simulink model "cars"  (Simulink 9.2)
settings: Solver=VariableStepAuto  StartTime=0  StopTime=100  FixedStep=0.1  MinStep=0.01  RelTol=1e-3  AbsTol=1e-5  EnableMultiTasking=on
settings Model: Creator=yoriyuki  LastModifiedBy=yoriyuki
settings SolverCC: AutoInsertRateTranBlk=on
settings DataIOCC: ExternalInput=[Throttle, Brake]  FinalStateName=SavePoint  InitialState=SavePoint  LimitDataPoints=off  SaveCompleteFinalSimState=on  SaveFormat=Dataset  SignalLoggingSaveFormat=Dataset  SaveOutput=off  SaveTime=off  StateSaveName=x  TimeSaveName=t  OutputSaveName=y
settings DebuggingCC: UnderspecifiedInitializationDetection=Simplified  MergeDetectMultiDrivingBlocksExec=error  FcnCallInpInsideContextMsg=error  AllowSymbolicDim=off  StateNameClashWarn=none
settings HardwareCC: ProdBitPerPointer=64  ProdBitPerSizeT=64  ProdBitPerPtrDiffT=64  ProdLargestAtomicFloat=Float  ProdIntDivRoundTo=Zero  ProdEndianess=LittleEndian  ProdWordSize=64  ProdHWDeviceType=Intel->x86-64 (Windows64)
settings ModelReferenceCC: PropagateSignalLabelsOutOfModel=on
settings GRTTargetCC: GeneratePreprocessorConditionals=Use local settings  CombineOutputUpdateFcns=on  GRTInterface=off
settings ConfigComp: CovShowResultsExplorer=off

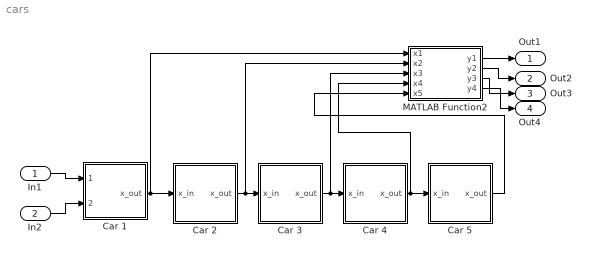
== system cars ==
  In1 : Inport
  In2 : Inport  Port=2
  Car 1 : Stateflow chart  TreatAsAtomicUnit=on
  Car 2 : Stateflow chart  TreatAsAtomicUnit=on
  Car 3 : Stateflow chart  TreatAsAtomicUnit=on
  Car 4 : Stateflow chart  TreatAsAtomicUnit=on
  Car 5 : Stateflow chart  TreatAsAtomicUnit=on
  MATLAB Function2 : MATLAB Function  TreatAsAtomicUnit=on
  Out1 : Outport
  Out2 : Outport  Port=2
  Out3 : Outport  Port=3
  Out4 : Outport  Port=4
  wires:
  Car 1/1(x_out) -> MATLAB Function2/1(x1), Car 2/1(x_in)
  Car 2/1(x_out) -> MATLAB Function2/2(x2), Car 3/1(x_in)
  Car 3/1(x_out) -> MATLAB Function2/3(x3), Car 4/1(x_in)
  Car 4/1(x_out) -> MATLAB Function2/4(x4), Car 5/1(x_in)
  Car 5/1(x_out) -> MATLAB Function2/5(x5)
  MATLAB Function2/1(y1) -> Out1/1
  MATLAB Function2/2(y2) -> Out2/1
  MATLAB Function2/3(y3) -> Out3/1
  MATLAB Function2/4(y4) -> Out4/1
  In1/1 -> Car 1/1(Throttle)
  In2/1 -> Car 1/2(Brake)

== stateflow chart Car 1 ==
  settings: updateMethod=CONTINUOUS
  state Run
    during:
    v_dot = -Throttle - Brake * v;
    x_dot = v;
    x_out = x;
  (default) -> Run
  data: Throttle input double; Brake input double; x local double =0; x_out output double; v local double =0
  data x settings: updateMethod=SF_CONTINUOUS_TIME_DATA
  data v settings: updateMethod=SF_CONTINUOUS_TIME_DATA

== stateflow chart Car 3 ==
  settings: updateMethod=CONTINUOUS
  state Chasing
    during:
    v_dot = 1;
    x_dot = -v;
    x_out = x;
  state Keeping
    during:
    x_dot = v;
    x_out = x;
  state Braking
    during:
    v_dot = -v;
    x_dot = -v;
    x_out = x;
  (default) -> Keeping
  Chasing -> Keeping : [x - x_in <= 10]
      | % [transition condition]{action}
  Keeping -> Chasing [order 1] : [x - x_in >=15]
  Braking -> Chasing : [x - x_in >= 20]
  Keeping -> Braking [order 2] : [x - x_in <=5]
  data: x_out output double; x local double =20; v local double =0; x_in input double
  data x settings: updateMethod=SF_CONTINUOUS_TIME_DATA
  data v settings: updateMethod=SF_CONTINUOUS_TIME_DATA
  data x_in settings: updateMethod=SF_CONTINUOUS_TIME_DATA

== stateflow chart Car 2 ==
  settings: updateMethod=CONTINUOUS
  state Chasing
    during:
    v_dot = 1;
    x_dot = -v;
    x_out = x;
  state Keeping
    during:
    x_dot = v;
    x_out = x;
  state Braking
    during:
    v_dot = -v;
    x_dot = -v;
    x_out = x;
  (default) -> Keeping
  Chasing -> Keeping : [x - x_in <= 10]
      | % [transition condition]{action}
  Keeping -> Chasing [order 1] : [x - x_in >=15]
  Braking -> Chasing : [x - x_in >= 20]
  Keeping -> Braking [order 2] : [x - x_in <=5]
  data: x_out output double; x local double =10; v local double =0; x_in input double
  data x settings: updateMethod=SF_CONTINUOUS_TIME_DATA
  data v settings: updateMethod=SF_CONTINUOUS_TIME_DATA
  data x_in settings: updateMethod=SF_CONTINUOUS_TIME_DATA

== stateflow chart Car 4 ==
  settings: updateMethod=CONTINUOUS
  state Chasing
    during:
    v_dot = 1;
    x_dot = -v;
    x_out = x;
  state Keeping
    during:
    x_dot = v;
    x_out = x;
  state Braking
    during:
    v_dot = -v;
    x_dot = -v;
    x_out = x;
  (default) -> Keeping
  Chasing -> Keeping : [x - x_in <= 10]
      | % [transition condition]{action}
  Keeping -> Chasing [order 1] : [x - x_in >=15]
  Braking -> Chasing : [x - x_in >= 20]
  Keeping -> Braking [order 2] : [x - x_in <=5]
  data: x_out output double; x local double =30; v local double =0; x_in input double
  data x settings: updateMethod=SF_CONTINUOUS_TIME_DATA
  data v settings: updateMethod=SF_CONTINUOUS_TIME_DATA
  data x_in settings: updateMethod=SF_CONTINUOUS_TIME_DATA

== stateflow chart Car 5 ==
  settings: updateMethod=CONTINUOUS
  state Keeping
    during:
    x_dot = v;
    x_out = x;
  state Chasing
    during:
    v_dot = 1;
    x_dot = -v;
    x_out = x;
  state Braking
    during:
    v_dot = -v;
    x_dot = -v;
    x_out = x;
  (default) -> Keeping
  Chasing -> Keeping : [x - x_in <= 10]
      | % [transition condition]{action}
  Keeping -> Chasing [order 1] : [x - x_in >=15]
  Braking -> Chasing : [x - x_in >= 20]
  Keeping -> Braking [order 2] : [x - x_in <=5]
  data: x_out output double; x local double =40; v local double =0; x_in input double
  data x settings: updateMethod=SF_CONTINUOUS_TIME_DATA
  data v settings: updateMethod=SF_CONTINUOUS_TIME_DATA
  data x_in settings: updateMethod=SF_CONTINUOUS_TIME_DATA

== matlab function MATLAB Function2 ==
  data: x1 input double; y1 output double; x2 input double; x3 input double; x4 input double; x5 input double; y2 output double; y3 output double; y4 output double
function [y1, y2, y3, y4] = diff(x1, x2, x3, x4, x5)
y1 = x2 - x1; 
y2 = x3 - x2; 
y3 = x4 - x3; 
y4 = x5 - x4;
